simulink model "s_c107m32k_vlbi"  (R2018a)
settings: Solver=VariableStepDiscrete  StartTime=0.0  StopTime=(2^15)*10  RelTol=1e-3
undefined symbols (not defined in the file): fft_stages, n_bits_xengs
libraries: xbsIndex_r4 x23049, casper_library_misc x45, xps_library x4, casper_library_scopes x3, simulink x2
(part 91 of 201)

== system s_c107m32k_vlbi/DDC/dec_fir_async2/fir_col_async6 ==
  real1 : Inport
  imag1 : Inport  Port=2
  real2 : Inport  Port=3
  imag2 : Inport  Port=4
  real3 : Inport  Port=5
  imag3 : Inport  Port=6
  real4 : Inport  Port=7
  imag4 : Inport  Port=8
  real5 : Inport  Port=9
  imag5 : Inport  Port=10
  real6 : Inport  Port=11
  imag6 : Inport  Port=12
  real7 : Inport  Port=13
  imag7 : Inport  Port=14
  real8 : Inport  Port=15
  imag8 : Inport  Port=16
  real9 : Inport  Port=17
  imag9 : Inport  Port=18
  real10 : Inport  Port=19
  imag10 : Inport  Port=20
  real11 : Inport  Port=21
  imag11 : Inport  Port=22
  real12 : Inport  Port=23
  imag12 : Inport  Port=24
  real13 : Inport  Port=25
  imag13 : Inport  Port=26
  real14 : Inport  Port=27
  imag14 : Inport  Port=28
  real15 : Inport  Port=29
  imag15 : Inport  Port=30
  real16 : Inport  Port=31
  imag16 : Inport  Port=32
  real_back1 : Inport  Port=33
  imag_back1 : Inport  Port=34
  real_back2 : Inport  Port=35
  imag_back2 : Inport  Port=36
  real_back3 : Inport  Port=37
  imag_back3 : Inport  Port=38
  real_back4 : Inport  Port=39
  imag_back4 : Inport  Port=40
  real_back5 : Inport  Port=41
  imag_back5 : Inport  Port=42
  real_back6 : Inport  Port=43
  imag_back6 : Inport  Port=44
  real_back7 : Inport  Port=45
  imag_back7 : Inport  Port=46
  real_back8 : Inport  Port=47
  imag_back8 : Inport  Port=48
  real_back9 : Inport  Port=49
  imag_back9 : Inport  Port=50
  real_back10 : Inport  Port=51
  imag_back10 : Inport  Port=52
  real_back11 : Inport  Port=53
  imag_back11 : Inport  Port=54
  real_back12 : Inport  Port=55
  imag_back12 : Inport  Port=56
  real_back13 : Inport  Port=57
  imag_back13 : Inport  Port=58
  real_back14 : Inport  Port=59
  imag_back14 : Inport  Port=60
  real_back15 : Inport  Port=61
  imag_back15 : Inport  Port=62
  real_back16 : Inport  Port=63
  imag_back16 : Inport  Port=64
  dv : Inport  Port=65
  adder_tree1 : Subsystem  AncestorBlock=casper_library_misc/adder_tree  mask(adder_tree){n_inputs=16, csp_latency=7, adder_imp=DSP48, first_stage_hdl=on, floating_point=off, dvalid_en=on, float_type=single, frac_width=0, exp_width=0}
      mask prompts: n_inputs "Number of Inputs"; csp_latency "Add Latency"; adder_imp "Adder implementation"; first_stage_hdl "Use behavioural HDL for first stage of adders"; floating_point "floating point"; float_type "float type"; frac_width "fraction length"; exp_width "exponent length"
      mask help:
      | Sums all inputs using a tree of adds and delays.
      |
      | Number of inputs: The number of inputs to the block to be summed
      | Add latency: The number of clock cycles to perform one addition (affects timing)..
      | Adder implementation: choice of fabric or DSP48E core, or behavioral HDL
      | Use behavioural HDL for first stage of adders: Causes the first stage of adders to be absorbed into DSP blocks if multipliers precede them (Virtex 5). Overrides Adder implementation
      mask init: same as s_c107m32k_vlbi/DDC/dec_fir_async/imag_sum
      settings: AttributesFormatString=latency 28
      mask Help: eval('xlWeb(''http://casper.berkeley.edu/wiki/Adder_tree'')')
      mask TypeOptions adder_imp: Behavioral | Fabric | DSP48
      mask Callback floating_point:
      | onoff = get_param(gcb, 'floating_point');
      | if strcmp(onoff,'on')
      |     enable_fixpt = 'off'
      |     set_param_state(gcb, 'float_type', 'on')
      | 
      |     f_type = get_param(gcb, 'float_type')
      |     if strcmp(f_type,'custom')
      |         set_param_state(gcb, 'exp_width', 'on')
      |         set_param_state(gcb, 'frac_width', 'on')
      |     else
      |         set_param_state(gcb, 'exp_width', 'off')
      |         set_param_state(gcb, 'frac_width', 'off')
      |     end
      | 
      | 
      | else
      |     enable_fixpt = 'on'
      |     set_param_state(gcb, 'float_type', 'off')
      |     set_param_state(gcb, 'exp_width', 'off')
      |     set_param_state(gcb, 'frac_width', 'off')
      | end
      mask TypeOptions float_type: single | custom
      mask Callback float_type:
      | f_type = get_param(gcb, 'float_type')
      | if strcmp(f_type,'custom')
      |     set_param_state(gcb, 'exp_width', 'on')
      |     set_param_state(gcb, 'frac_width', 'on')
      | else
      |     set_param_state(gcb, 'exp_width', 'off')
      |     set_param_state(gcb, 'frac_width', 'off')
      | end
  adder_tree2 : Subsystem  AncestorBlock=casper_library_misc/adder_tree  mask(adder_tree){n_inputs=16, csp_latency=7, adder_imp=DSP48, first_stage_hdl=on, floating_point=off, dvalid_en=on, float_type=single, frac_width=0, exp_width=0}
      mask prompts: n_inputs "Number of Inputs"; csp_latency "Add Latency"; adder_imp "Adder implementation"; first_stage_hdl "Use behavioural HDL for first stage of adders"; floating_point "floating point"; float_type "float type"; frac_width "fraction length"; exp_width "exponent length"
      mask help:
      | Sums all inputs using a tree of adds and delays.
      |
      | Number of inputs: The number of inputs to the block to be summed
      | Add latency: The number of clock cycles to perform one addition (affects timing)..
      | Adder implementation: choice of fabric or DSP48E core, or behavioral HDL
      | Use behavioural HDL for first stage of adders: Causes the first stage of adders to be absorbed into DSP blocks if multipliers precede them (Virtex 5). Overrides Adder implementation
      mask init: same as s_c107m32k_vlbi/DDC/dec_fir_async/imag_sum
      settings: AttributesFormatString=latency 28
      mask Help: eval('xlWeb(''http://casper.berkeley.edu/wiki/Adder_tree'')')
      mask TypeOptions adder_imp: Behavioral | Fabric | DSP48
      mask Callback floating_point:
      | onoff = get_param(gcb, 'floating_point');
      | if strcmp(onoff,'on')
      |     enable_fixpt = 'off'
      |     set_param_state(gcb, 'float_type', 'on')
      | 
      |     f_type = get_param(gcb, 'float_type')
      |     if strcmp(f_type,'custom')
      |         set_param_state(gcb, 'exp_width', 'on')
      |         set_param_state(gcb, 'frac_width', 'on')
      |     else
      |         set_param_state(gcb, 'exp_width', 'off')
      |         set_param_state(gcb, 'frac_width', 'off')
      |     end
      | 
      | 
      | else
      |     enable_fixpt = 'on'
      |     set_param_state(gcb, 'float_type', 'off')
      |     set_param_state(gcb, 'exp_width', 'off')
      |     set_param_state(gcb, 'frac_width', 'off')
      | end
      mask TypeOptions float_type: single | custom
      mask Callback float_type:
      | f_type = get_param(gcb, 'float_type')
      | if strcmp(f_type,'custom')
      |     set_param_state(gcb, 'exp_width', 'on')
      |     set_param_state(gcb, 'frac_width', 'on')
      | else
      |     set_param_state(gcb, 'exp_width', 'off')
      |     set_param_state(gcb, 'frac_width', 'off')
      | end
  c1 : xbsIndex_r4/Constant  const=1.0  gui_display_data_type=Fixed-point  arith_type=Signed (2's comp)  n_bits=16  bin_pt=14  preci_type=Single  exp_width=8  frac_width=24  explicit_period=on  period=1  equ=P=C  opselect=C  inp2=PCIN>>17  opr=+  inp1=P  carry=CIN  dbl_ovrd=off  block_type=constant
  c2 : xbsIndex_r4/Constant  const=1.0  gui_display_data_type=Fixed-point  arith_type=Signed (2's comp)  n_bits=16  bin_pt=14  preci_type=Single  exp_width=8  frac_width=24  explicit_period=on  period=1  equ=P=C  opselect=C  inp2=PCIN>>17  opr=+  inp1=P  carry=CIN  dbl_ovrd=off  block_type=constant
  fir_tap1 : Subsystem  AncestorBlock=casper_library_downconverter/fir_tap_async  mask(fir_tap_async){factor=-0.007637, add_latency=7, mult_latency=7, coeff_bit_width=18, coeff_bin_pt=17, async=on, dbl=on}
      mask prompts: add_latency "Add latency"; mult_latency "Mult latency"; coeff_bit_width "Coefficient bit width"; coeff_bin_pt "Coefficient binary point"; async "Asynchronous ops"; dbl "Double tap"
      mask help: Multiplies input data with factor specified.
      mask init:
      | fir_tap_async_init(gcb);
      mask Help: eval('xlWeb(''http://casper.berkeley.edu/wiki/Fir_tap'')')
  fir_tap10 : Subsystem  AncestorBlock=casper_library_downconverter/fir_tap_async  mask(fir_tap_async){factor=0.0062637, add_latency=7, mult_latency=7, coeff_bit_width=18, coeff_bin_pt=17, async=on, dbl=on}
      mask prompts: add_latency "Add latency"; mult_latency "Mult latency"; coeff_bit_width "Coefficient bit width"; coeff_bin_pt "Coefficient binary point"; async "Asynchronous ops"; dbl "Double tap"
      mask help: Multiplies input data with factor specified.
      mask init:
      | fir_tap_async_init(gcb);
      mask Help: eval('xlWeb(''http://casper.berkeley.edu/wiki/Fir_tap'')')
  fir_tap11 : Subsystem  AncestorBlock=casper_library_downconverter/fir_tap_async  mask(fir_tap_async){factor=0.0068665, add_latency=7, mult_latency=7, coeff_bit_width=18, coeff_bin_pt=17, async=on, dbl=on}
      mask prompts: add_latency "Add latency"; mult_latency "Mult latency"; coeff_bit_width "Coefficient bit width"; coeff_bin_pt "Coefficient binary point"; async "Asynchronous ops"; dbl "Double tap"
      mask help: Multiplies input data with factor specified.
      mask init:
      | fir_tap_async_init(gcb);
      mask Help: eval('xlWeb(''http://casper.berkeley.edu/wiki/Fir_tap'')')
  fir_tap12 : Subsystem  AncestorBlock=casper_library_downconverter/fir_tap_async  mask(fir_tap_async){factor=0.007225, add_latency=7, mult_latency=7, coeff_bit_width=18, coeff_bin_pt=17, async=on, dbl=on}
      mask prompts: add_latency "Add latency"; mult_latency "Mult latency"; coeff_bit_width "Coefficient bit width"; coeff_bin_pt "Coefficient binary point"; async "Asynchronous ops"; dbl "Double tap"
      mask help: Multiplies input data with factor specified.
      mask init:
      | fir_tap_async_init(gcb);
      mask Help: eval('xlWeb(''http://casper.berkeley.edu/wiki/Fir_tap'')')
  fir_tap13 : Subsystem  AncestorBlock=casper_library_downconverter/fir_tap_async  mask(fir_tap_async){factor=0.0073471, add_latency=7, mult_latency=7, coeff_bit_width=18, coeff_bin_pt=17, async=on, dbl=on}
      mask prompts: add_latency "Add latency"; mult_latency "Mult latency"; coeff_bit_width "Coefficient bit width"; coeff_bin_pt "Coefficient binary point"; async "Asynchronous ops"; dbl "Double tap"
      mask help: Multiplies input data with factor specified.
      mask init:
      | fir_tap_async_init(gcb);
      mask Help: eval('xlWeb(''http://casper.berkeley.edu/wiki/Fir_tap'')')
  fir_tap14 : Subsystem  AncestorBlock=casper_library_downconverter/fir_tap_async  mask(fir_tap_async){factor=0.0072403, add_latency=7, mult_latency=7, coeff_bit_width=18, coeff_bin_pt=17, async=on, dbl=on}
      mask prompts: add_latency "Add latency"; mult_latency "Mult latency"; coeff_bit_width "Coefficient bit width"; coeff_bin_pt "Coefficient binary point"; async "Asynchronous ops"; dbl "Double tap"
      mask help: Multiplies input data with factor specified.
      mask init:
      | fir_tap_async_init(gcb);
      mask Help: eval('xlWeb(''http://casper.berkeley.edu/wiki/Fir_tap'')')
  fir_tap15 : Subsystem  AncestorBlock=casper_library_downconverter/fir_tap_async  mask(fir_tap_async){factor=0.0069351, add_latency=7, mult_latency=7, coeff_bit_width=18, coeff_bin_pt=17, async=on, dbl=on}
      mask prompts: add_latency "Add latency"; mult_latency "Mult latency"; coeff_bit_width "Coefficient bit width"; coeff_bin_pt "Coefficient binary point"; async "Asynchronous ops"; dbl "Double tap"
      mask help: Multiplies input data with factor specified.
      mask init:
      | fir_tap_async_init(gcb);
      mask Help: eval('xlWeb(''http://casper.berkeley.edu/wiki/Fir_tap'')')
  fir_tap16 : Subsystem  AncestorBlock=casper_library_downconverter/fir_tap_async  mask(fir_tap_async){factor=0.0064468, add_latency=7, mult_latency=7, coeff_bit_width=18, coeff_bin_pt=17, async=on, dbl=on}
      mask prompts: add_latency "Add latency"; mult_latency "Mult latency"; coeff_bit_width "Coefficient bit width"; coeff_bin_pt "Coefficient binary point"; async "Asynchronous ops"; dbl "Double tap"
      mask help: Multiplies input data with factor specified.
      mask init:
      | fir_tap_async_init(gcb);
      mask Help: eval('xlWeb(''http://casper.berkeley.edu/wiki/Fir_tap'')')
  fir_tap2 : Subsystem  AncestorBlock=casper_library_downconverter/fir_tap_async  mask(fir_tap_async){factor=-0.0057373, add_latency=7, mult_latency=7, coeff_bit_width=18, coeff_bin_pt=17, async=on, dbl=on}
      mask prompts: add_latency "Add latency"; mult_latency "Mult latency"; coeff_bit_width "Coefficient bit width"; coeff_bin_pt "Coefficient binary point"; async "Asynchronous ops"; dbl "Double tap"
      mask help: Multiplies input data with factor specified.
      mask init:
      | fir_tap_async_init(gcb);
      mask Help: eval('xlWeb(''http://casper.berkeley.edu/wiki/Fir_tap'')')
  fir_tap3 : Subsystem  AncestorBlock=casper_library_downconverter/fir_tap_async  mask(fir_tap_async){factor=-0.0038147, add_latency=7, mult_latency=7, coeff_bit_width=18, coeff_bin_pt=17, async=on, dbl=on}
      mask prompts: add_latency "Add latency"; mult_latency "Mult latency"; coeff_bit_width "Coefficient bit width"; coeff_bin_pt "Coefficient binary point"; async "Asynchronous ops"; dbl "Double tap"
      mask help: Multiplies input data with factor specified.
      mask init:
      | fir_tap_async_init(gcb);
      mask Help: eval('xlWeb(''http://casper.berkeley.edu/wiki/Fir_tap'')')
  fir_tap4 : Subsystem  AncestorBlock=casper_library_downconverter/fir_tap_async  mask(fir_tap_async){factor=-0.0019302, add_latency=7, mult_latency=7, coeff_bit_width=18, coeff_bin_pt=17, async=on, dbl=on}
      mask prompts: add_latency "Add latency"; mult_latency "Mult latency"; coeff_bit_width "Coefficient bit width"; coeff_bin_pt "Coefficient binary point"; async "Asynchronous ops"; dbl "Double tap"
      mask help: Multiplies input data with factor specified.
      mask init:
      | fir_tap_async_init(gcb);
      mask Help: eval('xlWeb(''http://casper.berkeley.edu/wiki/Fir_tap'')')
  fir_tap5 : Subsystem  AncestorBlock=casper_library_downconverter/fir_tap_async  mask(fir_tap_async){factor=-0.00013733, add_latency=7, mult_latency=7, coeff_bit_width=18, coeff_bin_pt=17, async=on, dbl=on}
      mask prompts: add_latency "Add latency"; mult_latency "Mult latency"; coeff_bit_width "Coefficient bit width"; coeff_bin_pt "Coefficient binary point"; async "Asynchronous ops"; dbl "Double tap"
      mask help: Multiplies input data with factor specified.
      mask init:
      | fir_tap_async_init(gcb);
      mask Help: eval('xlWeb(''http://casper.berkeley.edu/wiki/Fir_tap'')')
  fir_tap6 : Subsystem  AncestorBlock=casper_library_downconverter/fir_tap_async  mask(fir_tap_async){factor=0.0015335, add_latency=7, mult_latency=7, coeff_bit_width=18, coeff_bin_pt=17, async=on, dbl=on}
      mask prompts: add_latency "Add latency"; mult_latency "Mult latency"; coeff_bit_width "Coefficient bit width"; coeff_bin_pt "Coefficient binary point"; async "Asynchronous ops"; dbl "Double tap"
      mask help: Multiplies input data with factor specified.
      mask init:
      | fir_tap_async_init(gcb);
      mask Help: eval('xlWeb(''http://casper.berkeley.edu/wiki/Fir_tap'')')
  fir_tap7 : Subsystem  AncestorBlock=casper_library_downconverter/fir_tap_async  mask(fir_tap_async){factor=0.0030365, add_latency=7, mult_latency=7, coeff_bit_width=18, coeff_bin_pt=17, async=on, dbl=on}
      mask prompts: add_latency "Add latency"; mult_latency "Mult latency"; coeff_bit_width "Coefficient bit width"; coeff_bin_pt "Coefficient binary point"; async "Asynchronous ops"; dbl "Double tap"
      mask help: Multiplies input data with factor specified.
      mask init:
      | fir_tap_async_init(gcb);
      mask Help: eval('xlWeb(''http://casper.berkeley.edu/wiki/Fir_tap'')')
  fir_tap8 : Subsystem  AncestorBlock=casper_library_downconverter/fir_tap_async  mask(fir_tap_async){factor=0.0043335, add_latency=7, mult_latency=7, coeff_bit_width=18, coeff_bin_pt=17, async=on, dbl=on}
      mask prompts: add_latency "Add latency"; mult_latency "Mult latency"; coeff_bit_width "Coefficient bit width"; coeff_bin_pt "Coefficient binary point"; async "Asynchronous ops"; dbl "Double tap"
      mask help: Multiplies input data with factor specified.
      mask init:
      | fir_tap_async_init(gcb);
      mask Help: eval('xlWeb(''http://casper.berkeley.edu/wiki/Fir_tap'')')
  fir_tap9 : Subsystem  AncestorBlock=casper_library_downconverter/fir_tap_async  mask(fir_tap_async){factor=0.0054169, add_latency=7, mult_latency=7, coeff_bit_width=18, coeff_bin_pt=17, async=on, dbl=on}
      mask prompts: add_latency "Add latency"; mult_latency "Mult latency"; coeff_bit_width "Coefficient bit width"; coeff_bin_pt "Coefficient binary point"; async "Asynchronous ops"; dbl "Double tap"
      mask help: Multiplies input data with factor specified.
      mask init:
      | fir_tap_async_init(gcb);
      mask Help: eval('xlWeb(''http://casper.berkeley.edu/wiki/Fir_tap'')')
  term1 : Terminator
  term2 : Terminator
  real_out1 : Outport
  imag_out1 : Outport  Port=2
  real_out2 : Outport  Port=3
  imag_out2 : Outport  Port=4
  real_out3 : Outport  Port=5
  imag_out3 : Outport  Port=6
  real_out4 : Outport  Port=7
  imag_out4 : Outport  Port=8
  real_out5 : Outport  Port=9
  imag_out5 : Outport  Port=10
  real_out6 : Outport  Port=11
  imag_out6 : Outport  Port=12
  real_out7 : Outport  Port=13
  imag_out7 : Outport  Port=14
  real_out8 : Outport  Port=15
  imag_out8 : Outport  Port=16
  real_out9 : Outport  Port=17
  imag_out9 : Outport  Port=18
  real_out10 : Outport  Port=19
  imag_out10 : Outport  Port=20
  real_out11 : Outport  Port=21
  imag_out11 : Outport  Port=22
  real_out12 : Outport  Port=23
  imag_out12 : Outport  Port=24
  real_out13 : Outport  Port=25
  imag_out13 : Outport  Port=26
  real_out14 : Outport  Port=27
  imag_out14 : Outport  Port=28
  real_out15 : Outport  Port=29
  imag_out15 : Outport  Port=30
  real_out16 : Outport  Port=31
  imag_out16 : Outport  Port=32
  real_back_out1 : Outport  Port=33
  imag_back_out1 : Outport  Port=34
  real_back_out2 : Outport  Port=35
  imag_back_out2 : Outport  Port=36
  real_back_out3 : Outport  Port=37
  imag_back_out3 : Outport  Port=38
  real_back_out4 : Outport  Port=39
  imag_back_out4 : Outport  Port=40
  real_back_out5 : Outport  Port=41
  imag_back_out5 : Outport  Port=42
  real_back_out6 : Outport  Port=43
  imag_back_out6 : Outport  Port=44
  real_back_out7 : Outport  Port=45
  imag_back_out7 : Outport  Port=46
  real_back_out8 : Outport  Port=47
  imag_back_out8 : Outport  Port=48
  real_back_out9 : Outport  Port=49
  imag_back_out9 : Outport  Port=50
  real_back_out10 : Outport  Port=51
  imag_back_out10 : Outport  Port=52
  real_back_out11 : Outport  Port=53
  imag_back_out11 : Outport  Port=54
  real_back_out12 : Outport  Port=55
  imag_back_out12 : Outport  Port=56
  real_back_out13 : Outport  Port=57
  imag_back_out13 : Outport  Port=58
  real_back_out14 : Outport  Port=59
  imag_back_out14 : Outport  Port=60
  real_back_out15 : Outport  Port=61
  imag_back_out15 : Outport  Port=62
  real_back_out16 : Outport  Port=63
  imag_back_out16 : Outport  Port=64
  real_sum : Outport  Port=65
  imag_sum : Outport  Port=66
  wires:
  dv/1 -> [dv_in], adder_tree1/1(dv_in), adder_tree2/1(dv_in)
  [dv_in] -> fir_tap1/5(dv_in)
  real1/1 -> fir_tap1/1(a)
  imag1/1 -> fir_tap1/2(b)
  real_back16/1 -> fir_tap1/3(c)
  imag_back16/1 -> fir_tap1/4(d)
  [dv_in] -> fir_tap2/5(dv_in)
  real2/1 -> fir_tap2/1(a)
  imag2/1 -> fir_tap2/2(b)
  real_back15/1 -> fir_tap2/3(c)
  imag_back15/1 -> fir_tap2/4(d)
  [dv_in] -> fir_tap3/5(dv_in)
  real3/1 -> fir_tap3/1(a)
  imag3/1 -> fir_tap3/2(b)
  real_back14/1 -> fir_tap3/3(c)
  imag_back14/1 -> fir_tap3/4(d)
  [dv_in] -> fir_tap4/5(dv_in)
  real4/1 -> fir_tap4/1(a)
  imag4/1 -> fir_tap4/2(b)
  real_back13/1 -> fir_tap4/3(c)
  imag_back13/1 -> fir_tap4/4(d)
  [dv_in] -> fir_tap5/5(dv_in)
  real5/1 -> fir_tap5/1(a)
  imag5/1 -> fir_tap5/2(b)
  real_back12/1 -> fir_tap5/3(c)
  imag_back12/1 -> fir_tap5/4(d)
  [dv_in] -> fir_tap6/5(dv_in)
  real6/1 -> fir_tap6/1(a)
  imag6/1 -> fir_tap6/2(b)
  real_back11/1 -> fir_tap6/3(c)
  imag_back11/1 -> fir_tap6/4(d)
  [dv_in] -> fir_tap7/5(dv_in)
  real7/1 -> fir_tap7/1(a)
  imag7/1 -> fir_tap7/2(b)
  real_back10/1 -> fir_tap7/3(c)
  imag_back10/1 -> fir_tap7/4(d)
  [dv_in] -> fir_tap8/5(dv_in)
  real8/1 -> fir_tap8/1(a)
  imag8/1 -> fir_tap8/2(b)
  real_back9/1 -> fir_tap8/3(c)
  imag_back9/1 -> fir_tap8/4(d)
  [dv_in] -> fir_tap9/5(dv_in)
  real9/1 -> fir_tap9/1(a)
  imag9/1 -> fir_tap9/2(b)
  real_back8/1 -> fir_tap9/3(c)
  imag_back8/1 -> fir_tap9/4(d)
  [dv_in] -> fir_tap10/5(dv_in)
  real10/1 -> fir_tap10/1(a)
  imag10/1 -> fir_tap10/2(b)
  real_back7/1 -> fir_tap10/3(c)
  imag_back7/1 -> fir_tap10/4(d)
  [dv_in] -> fir_tap11/5(dv_in)
  real11/1 -> fir_tap11/1(a)
  imag11/1 -> fir_tap11/2(b)
  real_back6/1 -> fir_tap11/3(c)
  imag_back6/1 -> fir_tap11/4(d)
  [dv_in] -> fir_tap12/5(dv_in)
  real12/1 -> fir_tap12/1(a)
  imag12/1 -> fir_tap12/2(b)
  real_back5/1 -> fir_tap12/3(c)
  imag_back5/1 -> fir_tap12/4(d)
  [dv_in] -> fir_tap13/5(dv_in)
  real13/1 -> fir_tap13/1(a)
  imag13/1 -> fir_tap13/2(b)
  real_back4/1 -> fir_tap13/3(c)
  imag_back4/1 -> fir_tap13/4(d)
  [dv_in] -> fir_tap14/5(dv_in)
  real14/1 -> fir_tap14/1(a)
  imag14/1 -> fir_tap14/2(b)
  real_back3/1 -> fir_tap14/3(c)
  imag_back3/1 -> fir_tap14/4(d)
  [dv_in] -> fir_tap15/5(dv_in)
  real15/1 -> fir_tap15/1(a)
  imag15/1 -> fir_tap15/2(b)
  real_back2/1 -> fir_tap15/3(c)
  imag_back2/1 -> fir_tap15/4(d)
  [dv_in] -> fir_tap16/5(dv_in)
  real16/1 -> fir_tap16/1(a)
  imag16/1 -> fir_tap16/2(b)
  real_back1/1 -> fir_tap16/3(c)
  imag_back1/1 -> fir_tap16/4(d)
  fir_tap1/1(a_out) -> real_out1/1
  fir_tap1/2(b_out) -> imag_out1/1
  fir_tap1/3(c_out) -> real_back_out16/1
  fir_tap1/4(d_out) -> imag_back_out16/1
  fir_tap2/1(a_out) -> real_out2/1
  fir_tap2/2(b_out) -> imag_out2/1
  fir_tap2/3(c_out) -> real_back_out15/1
  fir_tap2/4(d_out) -> imag_back_out15/1
  fir_tap3/1(a_out) -> real_out3/1
  fir_tap3/2(b_out) -> imag_out3/1
  fir_tap3/3(c_out) -> real_back_out14/1
  fir_tap3/4(d_out) -> imag_back_out14/1
  fir_tap4/1(a_out) -> real_out4/1
  fir_tap4/2(b_out) -> imag_out4/1
  fir_tap4/3(c_out) -> real_back_out13/1
  fir_tap4/4(d_out) -> imag_back_out13/1
  fir_tap5/1(a_out) -> real_out5/1
  fir_tap5/2(b_out) -> imag_out5/1
  fir_tap5/3(c_out) -> real_back_out12/1
  fir_tap5/4(d_out) -> imag_back_out12/1
  fir_tap6/1(a_out) -> real_out6/1
  fir_tap6/2(b_out) -> imag_out6/1
  fir_tap6/3(c_out) -> real_back_out11/1
  fir_tap6/4(d_out) -> imag_back_out11/1
  fir_tap7/1(a_out) -> real_out7/1
  fir_tap7/2(b_out) -> imag_out7/1
  fir_tap7/3(c_out) -> real_back_out10/1
  fir_tap7/4(d_out) -> imag_back_out10/1
  fir_tap8/1(a_out) -> real_out8/1
  fir_tap8/2(b_out) -> imag_out8/1
  fir_tap8/3(c_out) -> real_back_out9/1
  fir_tap8/4(d_out) -> imag_back_out9/1
  fir_tap9/1(a_out) -> real_out9/1
  fir_tap9/2(b_out) -> imag_out9/1
  fir_tap9/3(c_out) -> real_back_out8/1
  fir_tap9/4(d_out) -> imag_back_out8/1
  fir_tap10/1(a_out) -> real_out10/1
  fir_tap10/2(b_out) -> imag_out10/1
  fir_tap10/3(c_out) -> real_back_out7/1
  fir_tap10/4(d_out) -> imag_back_out7/1
  fir_tap11/1(a_out) -> real_out11/1
  fir_tap11/2(b_out) -> imag_out11/1
  fir_tap11/3(c_out) -> real_back_out6/1
  fir_tap11/4(d_out) -> imag_back_out6/1
  fir_tap12/1(a_out) -> real_out12/1
  fir_tap12/2(b_out) -> imag_out12/1
  fir_tap12/3(c_out) -> real_back_out5/1
  fir_tap12/4(d_out) -> imag_back_out5/1
  fir_tap13/1(a_out) -> real_out13/1
  fir_tap13/2(b_out) -> imag_out13/1
  fir_tap13/3(c_out) -> real_back_out4/1
  fir_tap13/4(d_out) -> imag_back_out4/1
  fir_tap14/1(a_out) -> real_out14/1
  fir_tap14/2(b_out) -> imag_out14/1
  fir_tap14/3(c_out) -> real_back_out3/1
  fir_tap14/4(d_out) -> imag_back_out3/1
  fir_tap15/1(a_out) -> real_out15/1
  fir_tap15/2(b_out) -> imag_out15/1
  fir_tap15/3(c_out) -> real_back_out2/1
  fir_tap15/4(d_out) -> imag_back_out2/1
  fir_tap16/1(a_out) -> real_out16/1
  fir_tap16/2(b_out) -> imag_out16/1
  fir_tap16/3(c_out) -> real_back_out1/1
  fir_tap16/4(d_out) -> imag_back_out1/1
  adder_tree1/1(sync_out) -> term1/1
  adder_tree2/1(sync_out) -> term2/1
  c1/1 -> adder_tree1/2(sync)
  c2/1 -> adder_tree2/2(sync)
  adder_tree1/2(dout) -> real_sum/1
  adder_tree2/2(dout) -> imag_sum/1
  fir_tap1/5(real) -> adder_tree1/3(din1)
  fir_tap1/6(imag) -> adder_tree2/3(din1)
  fir_tap2/5(real) -> adder_tree1/4(din2)
  fir_tap2/6(imag) -> adder_tree2/4(din2)
  fir_tap3/5(real) -> adder_tree1/5(din3)
  fir_tap3/6(imag) -> adder_tree2/5(din3)
  fir_tap4/5(real) -> adder_tree1/6(din4)
  fir_tap4/6(imag) -> adder_tree2/6(din4)
  fir_tap5/5(real) -> adder_tree1/7(din5)
  fir_tap5/6(imag) -> adder_tree2/7(din5)
  fir_tap6/5(real) -> adder_tree1/8(din6)
  fir_tap6/6(imag) -> adder_tree2/8(din6)
  fir_tap7/5(real) -> adder_tree1/9(din7)
  fir_tap7/6(imag) -> adder_tree2/9(din7)
  fir_tap8/5(real) -> adder_tree1/10(din8)
  fir_tap8/6(imag) -> adder_tree2/10(din8)
  fir_tap9/5(real) -> adder_tree1/11(din9)
  fir_tap9/6(imag) -> adder_tree2/11(din9)
  fir_tap10/5(real) -> adder_tree1/12(din10)
  fir_tap10/6(imag) -> adder_tree2/12(din10)
  fir_tap11/5(real) -> adder_tree1/13(din11)
  fir_tap11/6(imag) -> adder_tree2/13(din11)
  fir_tap12/5(real) -> adder_tree1/14(din12)
  fir_tap12/6(imag) -> adder_tree2/14(din12)
  fir_tap13/5(real) -> adder_tree1/15(din13)
  fir_tap13/6(imag) -> adder_tree2/15(din13)
  fir_tap14/5(real) -> adder_tree1/16(din14)
  fir_tap14/6(imag) -> adder_tree2/16(din14)
  fir_tap15/5(real) -> adder_tree1/17(din15)
  fir_tap15/6(imag) -> adder_tree2/17(din15)
  fir_tap16/5(real) -> adder_tree1/18(din16)
  fir_tap16/6(imag) -> adder_tree2/18(din16)
